simulink model "NPC_SHM"  (R2024b)
settings: Solver=VariableStepAuto  StartTime=0.0  StopTime=0.30  RelTol=1e-3
values from neighbouring files (symbols this model uses):
  C1 = 470e-6    (= 0.00047)    [nonideal_model_init.m]
  C2 = 470e-6    (= 0.00047)    [nonideal_model_init.m]
  Td = 2e-6    (= 2e-06)    [nonideal_model_init.m]
  theta_deg = [4.323113 6.926852 21.464615 27.313345 32.230475 39.919268 44.218853 46.360690 50.066649 59.402712 61.055868 63.820445 67.679385 81.809510 86.375605]    [nonideal_model_init.m]
libraries: spsDiodeLib x19, spsIGBTLib x12, spsSeriesRLCBranchLib x6, spsCurrentMeasurementLib x3, spsVoltageMeasurementLib x3, spsDCVoltageSourceLib x1, spspowerguiLib x1
settings Model: Creator=medos  LastModifiedBy=medos

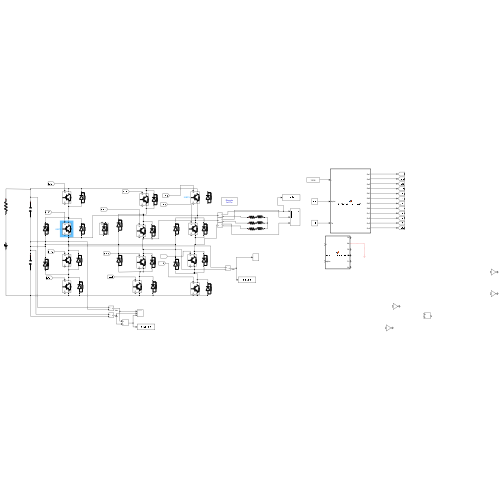
[thumbnail: Simulink's stored preview of the top-level diagram]
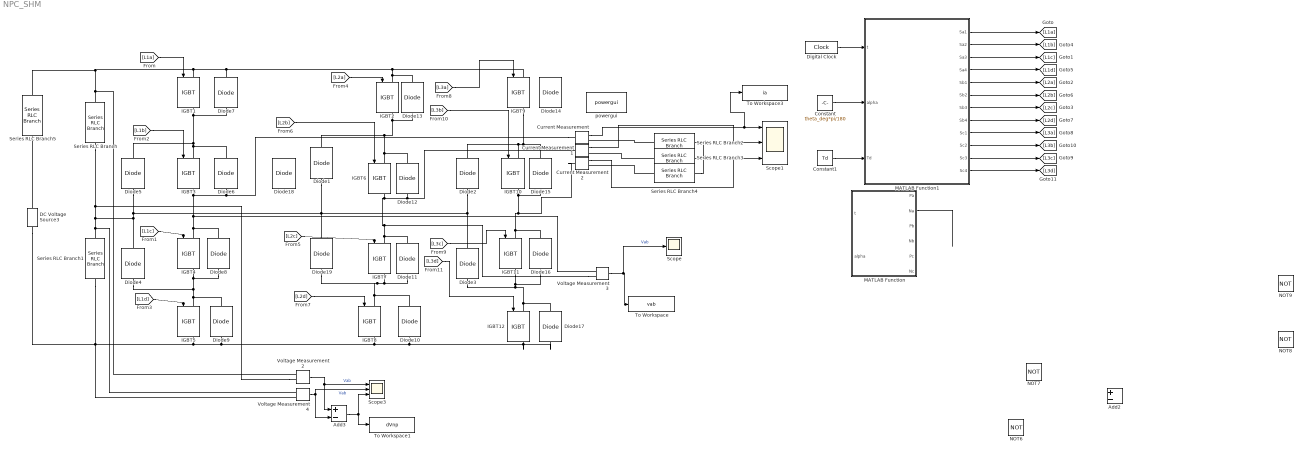
== system NPC_SHM ==
  Add2 : Sum  Inputs=+-
  Add3 : Sum  Inputs=+-
  Constant : Constant  Value=theta_deg*pi/180  SampleTime=-1
  Constant1 : Constant  Value=Td  SampleTime=-1
  Current Measurement : spsCurrentMeasurementLib/Current Measurement  PhasorSimulation=off  OutputType=Complex  PSBequivalent=0
  Current Measurement1 : spsCurrentMeasurementLib/Current Measurement  PhasorSimulation=off  OutputType=Complex  PSBequivalent=0
  Current Measurement2 : spsCurrentMeasurementLib/Current Measurement  PhasorSimulation=off  OutputType=Complex  PSBequivalent=0
  DC Voltage Source3 : spsDCVoltageSourceLib/DC Voltage Source  Amplitude=800  Measurements=None
  Digital Clock : DigitalClock  SampleTime=1e-6
  Diode{1..5,19} (6 alike) : spsDiodeLib/Diode  Ron=0.001  Lon=0  Vf=0.8  IC=0  UseSnubber=0  Rs=500  Cs=250e-9  Measurements=off
  Diode{6..17} (12 alike) : spsDiodeLib/Diode  Ron=Ron  Lon=0  Vf=Vfd  IC=0  UseSnubber=0  Rs=Rs  Cs=Cs  Measurements=off
  Diode18 : spsDiodeLib/Diode  Ron=0.001  Lon=0  Vf=0.8  IC=0  UseSnubber=0  Rs=500  Cs=250e-9  Measurements=on
  IGBT{1..12} (12 alike) : spsIGBTLib/IGBT  Ron=Ron  Lon=0  Vf=Vf  Tf=1e-6  Tt=2e-6  IC=0  Rs=Rs  Cs=Cs  Measurements=on
  MATLAB Function : MATLAB Function  TreatAsAtomicUnit=on
  MATLAB Function1 : MATLAB Function  TreatAsAtomicUnit=on
  NOT{6..9} (4 alike) : Logic  Operator=NOT  IconShape=distinctive  AllPortsSameDT=off  OutDataTypeStr=boolean
  Scope : Scope
  Scope1 : Scope  NumInputPorts=3
  Scope3 : Scope  NumInputPorts=3
  Series RLC Branch : spsSeriesRLCBranchLib/Series RLC Branch  LConnTagsString=__new0  RConnTagsString=__new0  BranchType=C  Resistance=0.01  Inductance=1e-3  SetiL0=off  InitialCurrent=0  Capacitance=C1  Setx0=on  InitialVoltage=VC1_0  Measurements=None
  Series RLC Branch1 : spsSeriesRLCBranchLib/Series RLC Branch  LConnTagsString=__new0  RConnTagsString=__new0  BranchType=C  Resistance=0.01  Inductance=1e-3  SetiL0=off  InitialCurrent=0  Capacitance=C2  Setx0=on  InitialVoltage=VC2_0  Measurements=None
  Series RLC Branch2 : spsSeriesRLCBranchLib/Series RLC Branch  LConnTagsString=__new0  RConnTagsString=__new0  BranchType=RL  Resistance=80  Inductance=25e-3  SetiL0=off  InitialCurrent=0  Capacitance=1e-6  Setx0=off  InitialVoltage=0  Measurements=None
  Series RLC Branch3 : spsSeriesRLCBranchLib/Series RLC Branch  LConnTagsString=__new0  RConnTagsString=__new0  BranchType=RL  Resistance=80  Inductance=25e-3  SetiL0=off  InitialCurrent=0  Capacitance=1e-6  Setx0=off  InitialVoltage=0  Measurements=None
  Series RLC Branch4 : spsSeriesRLCBranchLib/Series RLC Branch  LConnTagsString=__new0  RConnTagsString=__new0  BranchType=RL  Resistance=80  Inductance=25e-3  SetiL0=off  InitialCurrent=0  Capacitance=1e-6  Setx0=off  InitialVoltage=0  Measurements=None
  Series RLC Branch5 : spsSeriesRLCBranchLib/Series RLC Branch  LConnTagsString=__new0  RConnTagsString=__new0  BranchType=R  Resistance=0.0001  Inductance=1e-3  SetiL0=off  InitialCurrent=0  Capacitance=470e-6  Setx0=off  InitialVoltage=0  Measurements=None
  To Workspace : ToWorkspace  VariableName=vab  SaveFormat=Timeseries  SampleTime=-1
  To Workspace1 : ToWorkspace  VariableName=dVnp  SaveFormat=Timeseries  SampleTime=-1
  To Workspace3 : ToWorkspace  VariableName=ia  SaveFormat=Timeseries  SampleTime=-1
  Voltage Measurement2 : spsVoltageMeasurementLib/Voltage Measurement  PhasorSimulation=off  OutputType=Complex  PSBequivalent=0
  Voltage Measurement3 : spsVoltageMeasurementLib/Voltage Measurement  PhasorSimulation=off  OutputType=Complex  PSBequivalent=0
  Voltage Measurement4 : spsVoltageMeasurementLib/Voltage Measurement  PhasorSimulation=off  OutputType=Complex  PSBequivalent=0
  powergui : spspowerguiLib/powergui  Priority=1  SimulationMode=Discrete  SampleTime=1e-7  frequency=50  Iterations=50  frequencyindice=0  Pbase=100e6  ErrMax=1e-4  UnitsV=kV  UnitsW=MW  buscounter=0  FunctionMessages=off  echomessages=off  EnableUseOfTLC=off  CurrentSourceSwitches=off  DisableSnubberDevices=off  DisableRonSwitches=off  DisableVfSwitches=off  DisplayEquations=off  AutomaticDiscreteSolvers=off  SolverType=Tustin/Backward Euler (TBE)  Interpol=off  ExternalGateDelay=off  methode=off  Ts=100  x0status=blocks  SPID=on  SwTol=0  HookPort=off  NonlinearTolerance=1e-4  nMaxIteration=100  ContinueOnMaxIteration=off  RestoreLinks=warning  ResistiveCurrentMeasurement=off  Frange=[0:2:500]  Ylog=off  Xlog=on  ShowGrid=off  save=off  variable=ZData  structure=0  ZoomFFT=off  StartTime=0.0  cycles=1  DisplayStyle=1  fundamental=60  FreqAxis=off  MaxFrequency=1000  frequencyindicesteady=1  RmsSteady=1  display=off
  wires:
  [L2a] -> IGBT2/1
  [L2b] -> IGBT6/1
  [L2d] -> IGBT8/1
  [L1b] -> IGBT3/1
  [L3c] -> IGBT11/1
  [L1a] -> IGBT1/1
  [L1d] -> IGBT5/1
  [L2c] -> IGBT7/1
  [L3a] -> IGBT9/1
  Current Measurement2/1 -> Scope1/3
  MATLAB Function/2(Na) -> ?
  Current Measurement/1 -> To Workspace3/1, Scope1/1
  Current Measurement1/1 -> Scope1/2
  Voltage Measurement2/1 -> Add3/1, Scope3/1  "Vab"
  Add3/1 -> Scope3/3, To Workspace1/1
  [L3b] -> IGBT10/1
  [L3d] -> IGBT12/1
  [L1c] -> IGBT4/1
  Voltage Measurement4/1 -> Add3/2, Scope3/2  "Vab"
  Voltage Measurement3/1 -> Scope/1, To Workspace/1  "Vab"
  MATLAB Function1/12(Sc4) -> [L3d]
  MATLAB Function1/1(Sa1) -> [L1a]
  MATLAB Function1/2(Sa2) -> [L1b]
  MATLAB Function1/3(Sa3) -> [L1c]
  MATLAB Function1/4(Sa4) -> [L1d]
  MATLAB Function1/5(Sb1) -> [L2a]
  MATLAB Function1/6(Sb2) -> [L2b]
  MATLAB Function1/7(Sb3) -> [L2c]
  MATLAB Function1/8(Sb4) -> [L2d]
  MATLAB Function1/9(Sc1) -> [L3a]
  MATLAB Function1/10(Sc2) -> [L3b]
  MATLAB Function1/11(Sc3) -> [L3c]
  Digital Clock/1 -> MATLAB Function1/1(t)
  Constant/1 -> MATLAB Function1/2(alpha)
  Constant1/1 -> MATLAB Function1/3(Td)
  connections:
  IGBT5/RConn1 -- Series RLC Branch1/RConn1 -- Voltage Measurement4/LConn2 -- DC Voltage Source3/LConn1 -- Diode9/LConn1 -- Diode10/LConn1 -- Diode17/LConn1 -- IGBT12/RConn1 -- IGBT8/RConn1
  IGBT9/RConn1 -- Diode2/RConn1 -- IGBT10/LConn1 -- Diode15/RConn1
  Series RLC Branch3/RConn1 -- Series RLC Branch2/RConn1 -- Series RLC Branch4/RConn1
  IGBT1/RConn1 -- Diode7/LConn1 -- Diode5/RConn1 -- Diode6/RConn1 -- IGBT3/LConn1
  IGBT4/RConn1 -- Diode8/LConn1 -- Diode4/LConn1 -- Diode9/RConn1 -- IGBT5/LConn1
  Current Measurement2/LConn1 -- Diode15/LConn1 -- IGBT10/RConn1 -- Diode16/RConn1 -- IGBT11/LConn1
  Voltage Measurement2/LConn2 -- Series RLC Branch/RConn1 -- Voltage Measurement4/LConn1 -- Series RLC Branch1/LConn1 -- Diode4/RConn1 -- Diode5/LConn1 -- Diode19/RConn1 -- Diode3/RConn1 -- Diode2/LConn1 -- Diode1/LConn1
  Series RLC Branch/LConn1 -- Voltage Measurement2/LConn1 -- Series RLC Branch5/LConn1 -- Diode7/RConn1 -- Diode13/RConn1 -- IGBT2/LConn1 -- IGBT9/LConn1 -- IGBT1/LConn1
  Current Measurement/LConn1 -- IGBT3/RConn1 -- Diode8/RConn1 -- IGBT4/LConn1 -- Voltage Measurement3/LConn1 -- Diode6/LConn1
  Diode1/RConn1 -- Diode12/RConn1 -- IGBT6/LConn1 -- Diode13/LConn1 -- IGBT2/RConn1
  IGBT11/RConn1 -- Diode16/LConn1 -- Diode3/LConn1 -- Diode17/RConn1 -- IGBT12/LConn1
  Voltage Measurement3/LConn2 -- Diode11/RConn1 -- IGBT7/LConn1 -- Diode12/LConn1 -- Current Measurement1/LConn1 -- IGBT6/RConn1
  Diode19/LConn1 -- Diode10/RConn1 -- IGBT8/LConn1 -- Diode11/LConn1 -- IGBT7/RConn1
  Series RLC Branch4/LConn1 -- Current Measurement2/RConn1
  Series RLC Branch2/LConn1 -- Current Measurement/RConn1
  DC Voltage Source3/RConn1 -- Series RLC Branch5/RConn1
  Series RLC Branch3/LConn1 -- Current Measurement1/RConn1

== matlab function NPC_SHM/MATLAB Function1 ==
  data: t input; Sa1 output; alpha input double size=[1 15]; Sa2 output; Sa3 output; Sa4 output; Sb1 output; Sb2 output; Td input; Sb3 output; Sb4 output; Sc1 output; Sc2 output; Sc3 output; Sc4 output
function [Sa1,Sa2,Sa3,Sa4,Sb1,Sb2,Sb3,Sb4,Sc1,Sc2,Sc3,Sc4] = shmpwm3ph_15_deadtime(t, alpha, Td)
%#codegen
alpha = sort(alpha(:)).';
f = 50;
w = 2*pi*f;
[Sa1,Sa2,Sa3,Sa4] = leg_gates(w, t, 0,      alpha, Td);
[Sb1,Sb2,Sb3,Sb4] = leg_gates(w, t, 2*pi/3, alpha, Td);
[Sc1,Sc2,Sc3,Sc4] = leg_gates(w, t, 4*pi/3, alpha, Td);
end

function [S1,S2,S3,S4] = leg_gates(w, t, phi, alpha, Td)
L0 = phase_level(w*t - phi,        alpha);   % commanded level now
L1 = phase_level(w*(t - Td) - phi, alpha);   % commanded level Td ago
[P0, N0] = level_to_PN(L0);
[P1, N1] = level_to_PN(L1);
% on only if commanded on now AND Td ago (turn-on delayed), off at once
S1 = P0 * P1;
S3 = (1 - P0) * (1 - P1);
S4 = N0 * N1;
S2 = (1 - N0) * (1 - N1);
end

function L = phase_level(theta, alpha)
theta = mod(theta, 2*pi);
if theta <= pi/2
    L = first_quarter_level(theta, alpha);
elseif theta <= pi
    L = first_quarter_level(pi - theta, alpha);
elseif theta <= 3*pi/2
    L = -first_quarter_level(theta - pi, alpha);
else
    L = -first_quarter_level(2*pi - theta, alpha);
end
end

function L = first_quarter_level(theta, alpha)
L = 0;
for k = 1:length(alpha)
    if theta >= alpha(k)
        L = 1 - L;
    else
        break;
    end
end
end

function [P, N] = level_to_PN(L)
if L > 0.5
    P = 1; N = 0;
elseif L < -0.5
    P = 0; N = 1;
else
    P = 0; N = 0;
end
end

== matlab function NPC_SHM/MATLAB Function ==
  data: t input; Pa output; alpha input double size=[1 15]; Na output; Pb output; Nb output; Pc output; Nc output
function [Pa, Na, Pb, Nb, Pc, Nc] = shmpwm3ph_15_standard_fixed(t, alpha)

alpha = sort(alpha(:)).';

f = 50;
w = 2*pi*f;

La = phase_level(w*t,          alpha);
Lb = phase_level(w*t - 2*pi/3, alpha);
Lc = phase_level(w*t - 4*pi/3, alpha);

[Pa, Na] = level_to_PN(La);
[Pb, Nb] = level_to_PN(Lb);
[Pc, Nc] = level_to_PN(Lc);

end


function L = phase_level(theta, alpha)

theta = mod(theta, 2*pi);

if theta <= pi/2
    L = first_quarter_level(theta, alpha);

elseif theta <= pi
    L = first_quarter_level(pi - theta, alpha);

elseif theta <= 3*pi/2
    L = -first_quarter_level(theta - pi, alpha);

else
    L = -first_quarter_level(2*pi - theta, alpha);
end

end


function L = first_quarter_level(theta, alpha)

% IMPORTANT:
% Standard waveform from the paper starts at 0 in the first quarter,
% then toggles 0/1 at every switching angle.
L = 0;

for k = 1:length(alpha)
    if theta >= alpha(k)
        L = 1 - L;   % toggle: 0->1->0->1...
    else
        break;
    end
end

end


function [P, N] = level_to_PN(L)

if L > 0.5
    P = 1; N = 0;
elseif L < -0.5
    P = 0; N = 1;
else
    P = 0; N = 0;
end

end
